simulink model "mcb_pmsm_foc_sensorless_f28069MLaunchPad"  (R2024a)
settings: Solver=FixedStepDiscrete  StartTime=0.0  StopTime=8  RelTol=1e-3  EnableMultiTasking=on
InitFcn:
  | mcb_pmsm_foc_sensorless_f28069MLaunchPad_datascript;
undefined symbols (not defined in the file): acceleration, Down, GPTRIP1SEL, GPTRIP2SEL, inverter, MAX_OL_NEG_SPD, MAX_OL_POS_SPD, MAX_OL_VD_LIMIT, MIN_CL_NEG_SPD, MIN_CL_POS_SPD, MIN_OL_VD_LIMIT, one_sec_tick, PI_params, pmsm, PU_System, RAMP_STEP_SIZE, target, Ts, Ts_motor, Ts_simulink, Ts_speed, two_sec_tick, TZ1, TZ2, Up
libraries: mcbcontrolslib x16, c2802xlib x5, simulink x4, c280xlib x4, slpidlib x3, mcbpositiondecoderlib x3, c2806xlib x3, mcbsensorlessestimatorlib x2, svdschedulerlib x2, mcbplantlib x1, autolibpmsmexterior x1
(part 3 of 3)

== system mcb_pmsm_foc_sensorless_f28069MLaunchPad/Hardware Init/Variant Subsystem/Code Generation/Calculate ADC Offset /For Iterator Subsystem/If Action Subsystem ==
  In1 : Inport
  In2 : Inport  Port=2
  Action Port : ActionPort
  Memory : Memory  InheritSampleTime=on
  Memory1 : Memory  InheritSampleTime=on
  Sum : Sum
  Sum1 : Sum
  Out1 : Outport
  Out2 : Outport  Port=2
  wires:
  In1/1 -> Sum/1
  Sum/1 -> Out1/1, Memory/1
  In2/1 -> Sum1/1
  Memory/1 -> Sum/2
  Sum1/1 -> Out2/1, Memory1/1
  Memory1/1 -> Sum1/2

== stateflow chart mcb_pmsm_foc_sensorless_f28069MLaunchPad/State Machine Handler/State Machine OL - CL ==
  state RunMode
    state PositiveSpeedRun
      state OpenLoopPosRun
        during:
        if(SpdCmd>MAX_OL_POS_SPD)
        SpdRef=MAX_OL_POS_SPD;
        else
        SpdRef=SpdCmd;
        end
      state PreparePosCLSwitch
        entry:
        Id0_out=Id0_in;
        SpdRef=MAX_OL_POS_SPD;
      state TransferToPosClosedLoop
        entry:
        EnClosedLoop=true;
        Id0_out=Id0_in;
        during:
        Id0_out = ComputeId0(Id0_out,RAMP_STEP_SIZE);
      state TransferToOpenLoop
        entry:
        SpdRef=MAX_OL_POS_SPD*1.03;
      state ClosedLoopPosRun
        entry:
        SpdRef=SpdCmd;
        Id0_out=0;
        during:
        SpdRef=SpdCmd;
      (junction 118) -> (junction 94) [order 1] : [SpdCmd>MAX_OL_POS_SPD]
      (junction 94) -> PreparePosCLSwitch [order 2] : [SpdRef<MAX_OL_POS_SPD]
      (junction 94) -> TransferToPosClosedLoop [order 1] : [SpdRef>=MAX_OL_POS_SPD]
      OpenLoopPosRun -> (junction 118)
      PreparePosCLSwitch -> TransferToPosClosedLoop : after(one_sec_tick,tick)
      TransferToPosClosedLoop -> ClosedLoopPosRun : after(two_sec_tick,tick)[Id0_out<=RAMP_STEP_SIZE]
      ClosedLoopPosRun -> TransferToOpenLoop : [SpdCmd<MIN_CL_POS_SPD]
    state InitOpenLoopRun
      entry:
      Enable=true;
      EnClosedLoop=false;
      during:
      if(SpdCmd>MAX_OL_POS_SPD)
      SpdRef=MAX_OL_POS_SPD;
      elseif (SpdCmd<MAX_OL_NEG_SPD)
      SpdRef=MAX_OL_NEG_SPD;
      else
      SpdRef=SpdCmd;
      end
      Id0_out=Id0_in;
    state Id0_out = ComputeId0(Id0_in,RAMP_STEP_SIZE) [function]
    state NegativeSpeedRun
      state OpenLoopNegRun
        during:
        if(SpdCmd<MAX_OL_NEG_SPD)
        SpdRef=MAX_OL_NEG_SPD;
        else
        SpdRef=SpdCmd;
        end
      state TransferToNegClosedLoop
        entry:
        EnClosedLoop=true;
        Id0_out=Id0_in;
        during:
        Id0_out = ComputeId0(Id0_out,RAMP_STEP_SIZE);
      state PrepareNegCLSwitch
        entry:
        Id0_out=Id0_in;
        SpdRef=MAX_OL_NEG_SPD;
      state TransferToOpenLoop_NEG
        entry:
        SpdRef=MAX_OL_NEG_SPD*1.03;
      state ClosedLoopRun_NEG
        entry:
        SpdRef=SpdCmd;
        Id0_out=0;
        during:
        SpdRef=SpdCmd;
      OpenLoopNegRun -> (junction 121)
      (junction 121) -> (junction 124) [order 2] : [SpdCmd<MAX_OL_NEG_SPD]
      (junction 124) -> TransferToNegClosedLoop [order 2] : [SpdRef<=MAX_OL_NEG_SPD]
      (junction 124) -> PrepareNegCLSwitch [order 1] : [SpdRef>MAX_OL_NEG_SPD]
      PrepareNegCLSwitch -> TransferToNegClosedLoop : after(one_sec_tick,tick)
      TransferToNegClosedLoop -> ClosedLoopRun_NEG : after(two_sec_tick,tick)[Id0_out<=RAMP_STEP_SIZE]
      ClosedLoopRun_NEG -> TransferToOpenLoop_NEG : [SpdCmd>MIN_CL_NEG_SPD]
    InitOpenLoopRun -> OpenLoopPosRun [order 1] : [SpdCmd > 0]
    (junction 118) -> OpenLoopNegRun [order 2] : [SpdCmd<0]
    (junction 121) -> OpenLoopPosRun [order 1] : [SpdCmd>0]
    (default) -> InitOpenLoopRun
    TransferToOpenLoop_NEG -> InitOpenLoopRun : after(one_sec_tick,tick)
    InitOpenLoopRun -> OpenLoopNegRun [order 2] : [SpdCmd<0]
    TransferToOpenLoop -> InitOpenLoopRun : after(one_sec_tick,tick)
  state Halt
    entry:
    Enable=false;
    SpdRef=0;
    EnClosedLoop=false;
  Halt -> RunMode : [Start==true && SpdCmd~=0]
  (default) -> Halt
  RunMode -> Halt : [Start==false || SpdCmd==0]
  data: Id0_in function_input dataType size=1; RAMP_STEP_SIZE function_input dataType size=1; Id0_out function_output; Enable output; EnClosedLoop output; SpdRef output; Start input; SpdCmd input; Id0_out output dataType; Id0_in input; one_sec_tick parameter; two_sec_tick parameter; RAMP_STEP_SIZE parameter dataType; MAX_OL_NEG_SPD parameter dataType; MIN_CL_NEG_SPD parameter dataType; MIN_CL_POS_SPD parameter dataType; MAX_OL_POS_SPD parameter dataType
